simulink model "chaine_gauss"  (R2023b)
settings: Solver=FixedStepDiscrete  StartTime=0.0  StopTime=100000  FixedStep=1  RelTol=1e-3
values from neighbouring files (symbols this model uses):
  A = P.A    [Parametres.m]
  graine = round(P.graine)    [Parametres.m]    (also in Partie2.m = P.graine; parametres_perso.m = mod(sum(c .* (1:numel(c)) * 31) + 7 * numel(c), 2^31 - 1))
  p1 = P.p1    [Parametres.m]    (also in Partie2.m)
  seuil = 0    [test_cod.m]    (also in test_ech.m; test_gauss.m = seuils(k); test_retard.m; test_unif.m = seuils(k))
  sigma = P.sigma    [Parametres.m]
settings Model: Creator=e2403517  LastModifiedBy=e2403517

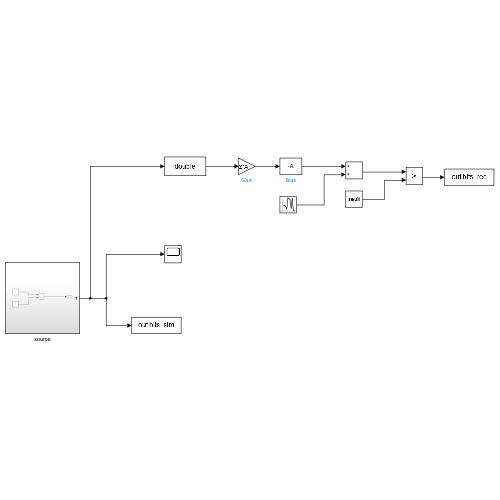
[thumbnail: Simulink's stored preview of the top-level diagram]
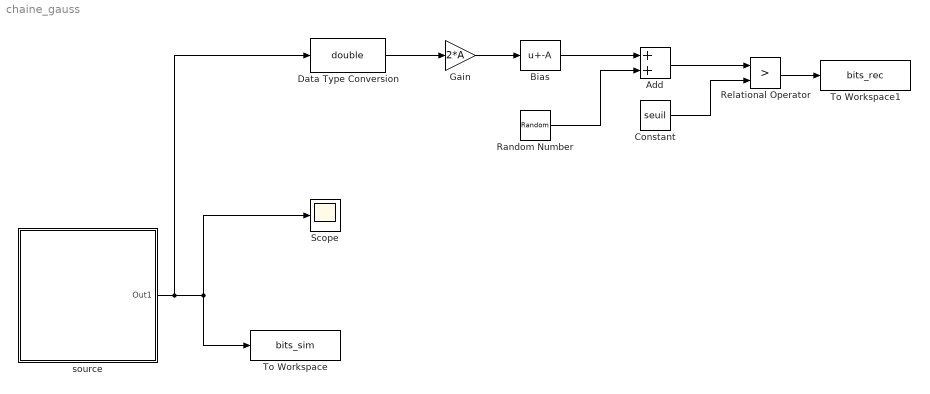
== system chaine_gauss ==
  Add : Sum
  Bias : Bias  Bias=-A  SaturateOnIntegerOverflow=off
  Constant : Constant  Value=seuil  SampleTime=1
  Data Type Conversion : DataTypeConversion  OutDataTypeStr=double  SaturateOnIntegerOverflow=off  RndMeth=Floor
  Gain : Gain  Gain=2*A
  Random Number : RandomNumber  Variance=sigma^2  Seed=graine+3  SampleTime=1
  Relational Operator : RelationalOperator  Operator=>  OutDataTypeStr=boolean  RndMeth=Simplest  InputSameDT=off
  Scope : Scope
  To Workspace : ToWorkspace  VariableName=bits_sim  SampleTime=1
  To Workspace1 : ToWorkspace  VariableName=bits_rec  SampleTime=1
  source : Subsystem
  wires:
  source/1(Out1) -> Data Type Conversion/1, Scope/1, To Workspace/1
  Data Type Conversion/1 -> Gain/1
  Gain/1 -> Bias/1
  Bias/1 -> Add/1
  Random Number/1 -> Add/2
  Add/1 -> Relational Operator/1
  Constant/1 -> Relational Operator/2
  Relational Operator/1 -> To Workspace1/1

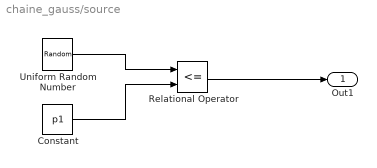
== system chaine_gauss/source ==
  Constant : Constant  Value=p1  SampleTime=1
  Relational Operator : RelationalOperator  Operator=<=  OutDataTypeStr=boolean  RndMeth=Simplest  InputSameDT=off
  Uniform Random Number : UniformRandomNumber  Minimum=0  Seed=graine  SampleTime=1
  Out1 : Outport
  wires:
  Uniform Random Number/1 -> Relational Operator/1
  Constant/1 -> Relational Operator/2
  Relational Operator/1 -> Out1/1
